simulink model "sumilink"  (R2026b)
settings: Solver=VariableStepAuto
settings Model: Creator=wpate  LastModifiedBy=wpate

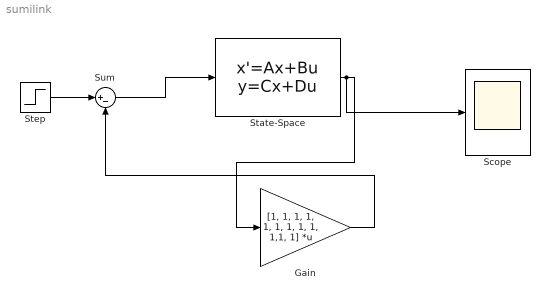
== system sumilink ==
  Gain : Gain  Gain=[1, 1, 1, 1, 1, 1, 1, 1, 1, 1,1, 1]  Multiplication=Matrix(K*u)
  Scope : Scope
      settings: ActiveDisplayYMinimum=-0.12374720056155289  ActiveDisplayYMaximum=1.1137247279017275
  State-Space : StateSpace  A=|  B=|  C=eye(12)  D=zeros(12,4)  InitialCondition=0
      A=|
      | [0 1 0 0 0 0 0 0 0 0 0 0;
      |  0 0 0 0 0 0 0 0 0 0 0 0;
      |  0 0 0 1 0 0 0 0 0 0 0 0; 0 0 0 0 0 0 -g 0 0 0 0 0;
      | 0 0 0 0 0 1 0 0 0 0 0 0;
      |  0 0 0 0 0 0 0 0 0 0 0 0;
      |  0 0 0 0 0 0 0 1 0 0 0 0;
      |  0 0 0 0 0 0 0 0 0 0 0 0;
      |  0 0 0 0 0 0 0 0 0 1 0 0;
      |  0 0 0 0 0 0 0 0 0 0 0 0;
      | 0 0 0 0 0 0 0 0 0 0 0 1;
      | 0 0 0 0 0 0 0 0 0 0 0 1];
      B=|
      | [0 0 0 0;
      |     0 g 0 0;
      |     0 0 0 0;
      |     0 g 0 0;
      |     0 0 0 0;
      |     m_0*g 0 0 0;
      |     0 0 0 0;
      |     0 0 0 0;
      |     0 0 0 0;
      |     0 -L/(m_0*g)*1/J_yy 0 0;
      |     0 0 0 0;
      |     0 0 0 0]
  Step : Step  FinalValue=[1,1,1,1]  SampleTime=0
  Sum : Sum  Inputs=|+-
  wires:
  Step/1 -> Sum/1
  State-Space/1 -> Scope/1, Gain/1
  Gain/1 -> Sum/2
  Sum/1 -> State-Space/1
